simulink model "Mission_Server_QDrone_Manual_Flight_FrSky_FA"  (Simulink 9.3)
settings: Solver=ode2  StartTime=0.0  StopTime=inf  FixedStep=0.001  RelTol=1e-3  EnableMultiTasking=on
InitFcn:
  | addpath(fileparts(get_param(bdroot,'FileName')));setup_project;
undefined symbols (not defined in the file or in its folder): datetime, Host, m, Mission_Server_, saved_data
libraries: quarc_library x16, simulink x5
settings Model: Creator=Admin  LastModifiedBy=user  SimulationMode=external  ExtModeTrigDuration=10000
settings SolverCC: PositivePriorityOrder=on
settings DataIOCC: SaveFormat=Dataset  SignalLoggingSaveFormat=Dataset
settings OptimizationCC: LifeSpan=auto
settings DebuggingCC: UnderspecifiedInitializationDetection=Simplified  MergeDetectMultiDrivingBlocksExec=error  FcnCallInpInsideContextMsg=error
settings HardwareCC: ProdBitPerPointer=64  ProdBitPerSizeT=64  ProdBitPerPtrDiffT=64  ProdLargestAtomicFloat=Float  ProdIntDivRoundTo=Zero  ProdEndianess=LittleEndian  ProdWordSize=64  ProdHWDeviceType=Intel->x86-64 (Windows64)
settings ModelReferenceCC: PropagateSignalLabelsOutOfModel=on
settings RTWCC: SystemTargetFile=quarc_win64.tlc  TemplateMakefile=quarc_default_tmf  Description=QUARC Win64 Target Using Toolchain  Toolchain=QUARC win64 | nmake (64-bit Windows)  BuildConfiguration=Faster Runs
settings STFCustomTargetCC: TargetPreCompLibLocation=C:\PROGRA~3\QUARC\lib\2019a\win64\release  ConcurrentExecutionCompliant=on  SystemTargetFile=quarc_win64.tlc
settings GRTTargetCC: TargetPreCompLibLocation=C:\PROGRA~3\QUARC\lib\2019a\win64\release  ParMdlRefBuildCompliant=off  CompOptLevelCompliant=off  MatFileLogging=off  CPPClassGenCompliant=off  UseToolchainInfoCompliant=off  ExtMode=on  ExtModeMexFile=quarc_comm  ExtModeMexArgs='-w -d %d -uri %u -URI_Host tcpip://192.168.2.5:18001'
settings ConfigComp: CovHtmlReporting=off

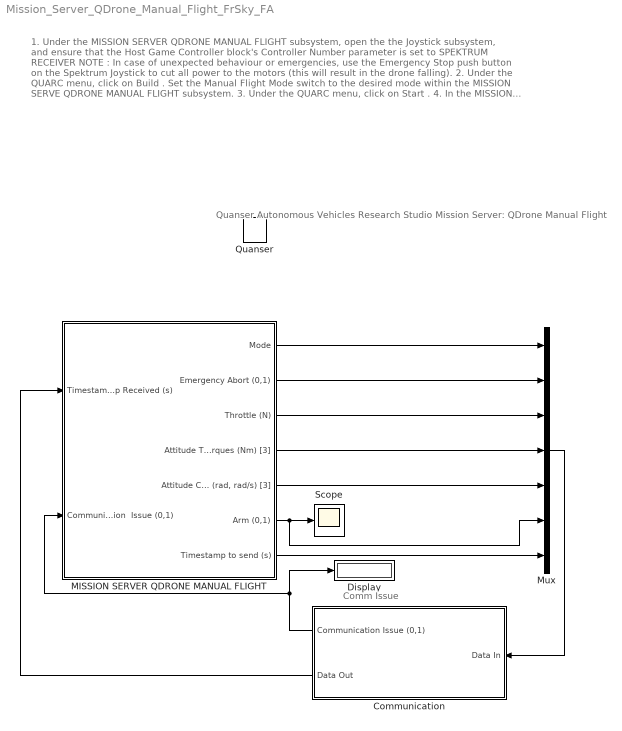
== system Mission_Server_QDrone_Manual_Flight_FrSky_FA ==
  note: Quanser Autonomous Vehicles Research Studio
      | Mission Server: QDrone Manual Flight
  note: 1. Under the MISSION SERVER QDRONE MANUAL FLIGHT subsystem, open the the Joystick subsystem, and ensure that the Host Game Controller block's Controller Number parameter is set to SPEKTRUM RECEIVER
      | NOTE : In case of unexpected behaviour or emergencies, use the Emergency Stop push button on the Spektrum Joystick to cut all power to the motors (this will result in the drone falling).
      | 2. Under the QUARC menu, click on Build . Set the Manual Flight Mode switch to the desired mode within the MISSION SERVE QDRONE MANUAL FLIGHT subsystem.
      | 3. Under the QUARC menu, click on Start .
      | 4. In the MISSION SERVER QDRONE MANUAL FLIGHT subsystem, ensure that the Joystick Issue display shows 0 (joystick must be powered ON with USB dongle attached to the PC).
      | 5. Ensure that the Stabilizer_QDrone.mdl model is running and that the Comm Issue display shows 0.
      | 6. Arm the drone by moving the Arm/Disarm toggle to the 2 position.
      | 7. Fly the drone manually. After landing, move the Arm/Disarm toggle to the 0 position to disarm the QDrone.
      | 8. Stop the Stabilizer_QDrone.mdl model first.
      | 9. Stop this model.
  note: Comm Issue
  Communication : Subsystem
  Display : Display
  MISSION SERVER QDRONE MANUAL FLIGHT : Subsystem
  Mux : Mux  Inputs=7
  Quanser : quarc_library/Logos/Quanser
  Scope : Scope
  wires:
  MISSION SERVER QDRONE MANUAL FLIGHT/7(Timestamp to send (s)) -> Mux/7
  MISSION SERVER QDRONE MANUAL FLIGHT/6(Arm (0,1)) -> Scope/1, Mux/6
  MISSION SERVER QDRONE MANUAL FLIGHT/5("Attitude Commands (rad, rad/s) [3]") -> Mux/5
  Communication/2(Data Out) -> MISSION SERVER QDRONE MANUAL FLIGHT/1(Timestamp Received (s))
  MISSION SERVER QDRONE MANUAL FLIGHT/4(Attitude Torques (Nm) [3]) -> Mux/4
  MISSION SERVER QDRONE MANUAL FLIGHT/3(Throttle (N)) -> Mux/3
  MISSION SERVER QDRONE MANUAL FLIGHT/2(Emergency Abort (0,1)) -> Mux/2
  Mux/1 -> Communication/1(Data In)
  MISSION SERVER QDRONE MANUAL FLIGHT/1(Mode) -> Mux/1
  Communication/1(Communication Issue (0,1)) -> MISSION SERVER QDRONE MANUAL FLIGHT/2(Communication  Issue (0,1)), Display/1

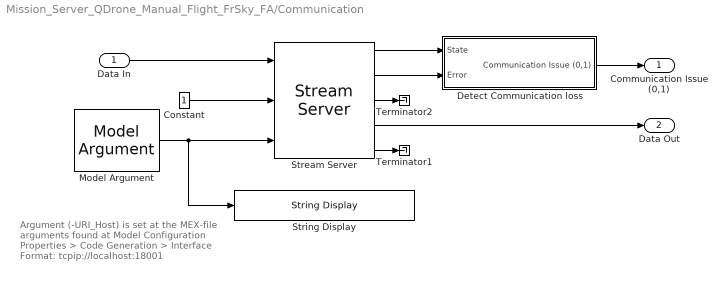
== system Mission_Server_QDrone_Manual_Flight_FrSky_FA/Communication ==
  note: Argument (-URI_Host) is set at the MEX-file arguments found at Model Configuration Properties > Code Generation > Interface
      |
      | Format:
      | tcpip://localhost:18001
  Data In : Inport
  Constant : Constant
  Detect Communication loss : Subsystem
  Model Argument : quarc_library/Sources/Signals/Model Argument  argument_name=URI_Host  has_value=on  data_type_mode=Specify via dialog  data_type=char  max_length=80  variable_size=off
      settings: AttributesFormatString=(-%<argument_name>)  SourceProductName=QUARC Targets
  Stream Server : quarc_library/Communications/Basic/Stream Server  uri_source=External input port  uri=tcpip://localhost:18877  apply_uri_to_all_configs=off  send_buffer_size=1460  receive_buffer_size=1460  byte_order=little endian (Intel - LSB first)  optimization=Minimum latency  send_options=Send most recent data  receive_options=Receive most recent data  default_value=zeros(1,2)  sample_time=qc_get_step_size  active=off  implementation=Use blocking I/O in a separate thread  send_fifo_size=1000  receive_fifo_size=1000  send_priority=0  receive_priority=0  send_dimensions=off  receive_dimensions=off  max_dimensions=-1  data_type=Inherited via back propagation  type_expr=BusObject
  "String Display " : quarc_library/Strings/String Display  alignment=center  display_mode=Single line  sample_time=-1  use_new=off
      settings: SourceProductName=QUARC Targets
  Terminator1 : Terminator
  Terminator2 : Terminator
  Communication Issue (0,1) : Outport
  Data Out : Outport  Port=2
  wires:
  Constant/1 -> Stream Server/2
  Data In/1 -> Stream Server/1
  Stream Server/3 -> Terminator2/1
  Stream Server/5 -> Terminator1/1
  Model Argument/1 -> "String Display "/1, Stream Server/3
  Stream Server/4 -> Data Out/1
  Stream Server/1 -> Detect Communication loss/1(State)
  Stream Server/2 -> Detect Communication loss/2(Error)
  Detect Communication loss/1(Communication Issue (0,1)) -> Communication Issue (0,1)/1

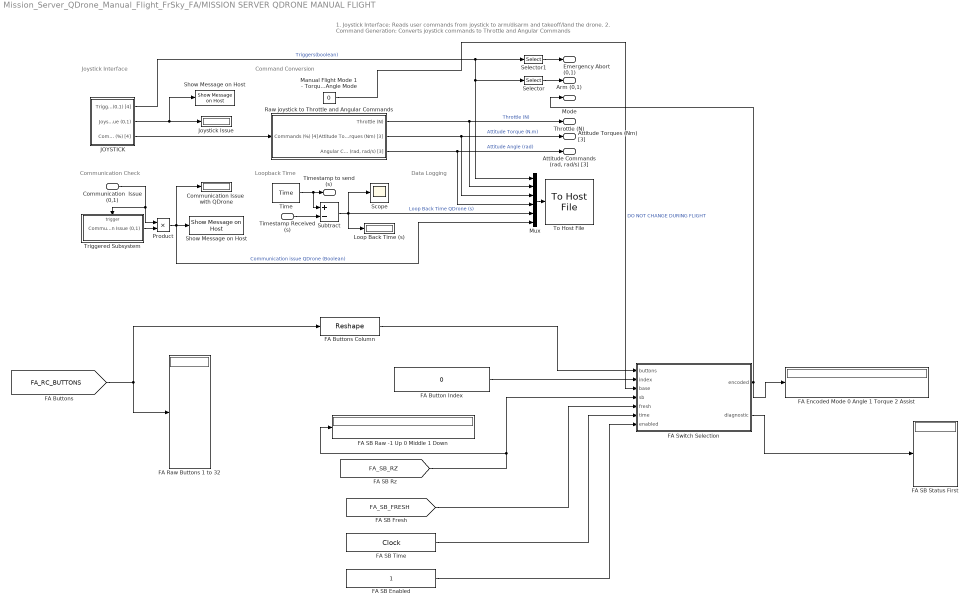
== system Mission_Server_QDrone_Manual_Flight_FrSky_FA/MISSION SERVER QDRONE MANUAL FLIGHT ==
  note: Loopback Time
  note: Command Conversion
  note: Data Logging
  note: Communication Check
  note: Joystick
      | Interface
  note: 1. Joystick Interface: Reads user commands from joystick to arm/disarm and takeoff/land the drone.
      | 2. Command Generation: Converts joystick commands to Throttle and Angular Commands
  Timestamp Received (s) : Inport
  Communication  Issue (0,1) : Inport  Port=2
  Communication Issue  with QDrone : Display
  FA Button Index : Constant  Value=0
  FA Buttons Column : Reshape  OutputDimensionality=Customize  OutputDimensions=[32 1]
  FA Encoded Mode 0 Angle 1 Torque 2 Assist : Display
  FA Raw Buttons 1 to 32 : Display
  FA SB Enabled : Constant
  FA SB Raw -1 Up 0 Middle 1 Down : Display
  FA SB Status First : Display
  FA SB Time : DigitalClock  SampleTime=0.001
  FA Switch Selection : MATLAB Function  TreatAsAtomicUnit=on
  JOYSTICK : Subsystem
  Joystick Issue : Display
  Loop Back Time (s) : Display
  "Manual Flight Mode 1 - Torque Mode,   0 - Angle Mode" : Constant  Value=0
  Mux : Mux  Inputs=6
  Product : Product
  Raw joystick to Throttle and Angular Commands : Subsystem
  Scope : Scope
  Selector : Selector  InputPortWidth=4  IndexOptions=Index vector (dialog)  Indices=[1]  OutputSizes=1
  Selector1 : Selector  InputPortWidth=4  IndexOptions=Index vector (dialog)  Indices=[3]  OutputSizes=1
  Show Message on Host : quarc_library/Sinks/Error Handling/Show Message on Host  message_type=Fixed error message  message_icon=Warning  message=Mission Server: Communication Issue with QDrone
      settings: AttributesFormatString="\"%<message>\""  SourceProductName=QUARC Targets
  "Show Message on Host " : quarc_library/Sinks/Error Handling/Show Message on Host  message_type=Fixed error message  message_icon=Warning  message=Mission Server: Joystick Disconnected
      settings: AttributesFormatString="\"%<message>\""  SourceProductName=QUARC Targets
  Subtract : Sum  Inputs=+-
  Time : quarc_library/Sources/Time/Time  time_source=Wall clock  sample_time=qc_get_step_size
  To Host File : quarc_library/Sinks/To Host/To Host File  file_name=saved_data/%m/Mission_Server_%{char(datetime)}.mat  variable_name=mission_server_data  decimation=1  sample_time=-1  file_format=MAT-file v.5  options=No header or footer  append=off  final_file_name=saved_data/Mission_Server_QDrone_Manual_Flight_FrSky_FA/Mission_Server_10-Nov-2026 20-24-39.mat  bitrate=2000000
  Triggered Subsystem : Subsystem  TreatAsAtomicUnit=on
  Mode : Outport
  Emergency Abort (0,1) : Outport  Port=2
  Throttle (N) : Outport  Port=3
  Attitude Torques (Nm) [3] : Outport  Port=4
  "Attitude Commands (rad, rad/s) [3]" : Outport  Port=5
  Arm (0,1) : Outport  Port=6
  Timestamp to send (s) : Outport  Port=7
  wires:
  Communication  Issue (0,1)/1 -> Product/1, Triggered Subsystem/Trigger
  JOYSTICK/2(Joystick Issue (0,1)) -> "Show Message on Host "/1, Joystick Issue/1
  JOYSTICK/3(Commands (%) [4]) -> Raw joystick to Throttle and Angular Commands/1(Commands (%) [4])
  JOYSTICK/1(Triggers (0,1) [4]) -> Selector1/1, Selector/1, Mux/1  "Triggers(boolean)"
  Time/1 -> Subtract/1, Timestamp to send (s)/1
  Timestamp Received (s)/1 -> Subtract/2
  Subtract/1 -> Loop Back Time (s)/1, Scope/1, Mux/5  "Loop Back Time QDrone (s)"
  Triggered Subsystem/1(Communication Issue (0,1)) -> Product/2
  Product/1 -> Communication Issue  with QDrone/1, Show Message on Host/1, Mux/6  "Communication issue QDrone (Boolean)"
  Mux/1 -> To Host File/1
  Selector/1 -> Arm (0,1)/1
  Selector1/1 -> Emergency Abort (0,1)/1
  Raw joystick to Throttle and Angular Commands/3("Angular Commands (rad, rad/s) [3]") -> "Attitude Commands (rad, rad/s) [3]"/1, Mux/4  "Attitude Angle (rad)"
  Raw joystick to Throttle and Angular Commands/1(Throttle (N)) -> Throttle (N)/1, Mux/2  "Throttle (N)"
  Raw joystick to Throttle and Angular Commands/2(Attitude Torques (Nm) [3]) -> Attitude Torques (Nm) [3]/1, Mux/3  "Attitude Torque (N.m)"
  "Manual Flight Mode 1 - Torque Mode,   0 - Angle Mode"/1 -> FA Switch Selection/3(base)  "DO NOT CHANGE DURING FLIGHT"
  [FA_RC_BUTTONS] -> FA Raw Buttons 1 to 32/1, FA Buttons Column/1
  FA Buttons Column/1 -> FA Switch Selection/1(buttons)
  FA Button Index/1 -> FA Switch Selection/2(index)
  FA Switch Selection/1(encoded) -> FA Encoded Mode 0 Angle 1 Torque 2 Assist/1, Mode/1
  [FA_SB_RZ] -> FA SB Raw -1 Up 0 Middle 1 Down/1, FA Switch Selection/4(sb)
  [FA_SB_FRESH] -> FA Switch Selection/5(fresh)
  FA SB Time/1 -> FA Switch Selection/6(time)
  FA SB Enabled/1 -> FA Switch Selection/7(enabled)
  FA Switch Selection/2(diagnostic) -> FA SB Status First/1

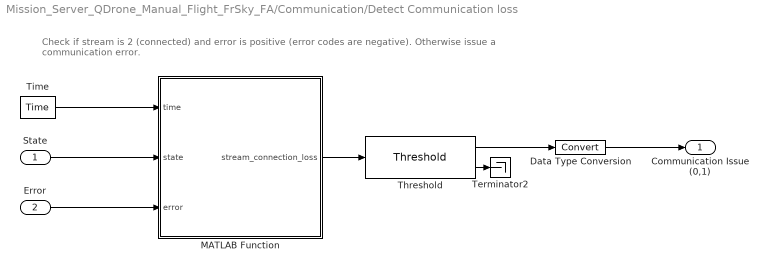
== system Mission_Server_QDrone_Manual_Flight_FrSky_FA/Communication/Detect Communication loss ==
  note: Check if stream is 2 (connected) and error is positive (error codes are negative). Otherwise issue a communication error.
  State : Inport
  Error : Inport  Port=2
  Data Type Conversion : DataTypeConversion
  MATLAB Function : MATLAB Function  TreatAsAtomicUnit=on
  Terminator2 : Terminator
  Threshold : quarc_library/Discontinuities/Threshold  operator=>=  param_src=Specify via dialog  threshold=0.5  duration=0.1
      settings: SourceProductName=QUARC Targets
  Time : quarc_library/Sources/Time/Time  time_source=Wall clock  sample_time=qc_get_step_size
  Communication Issue (0,1) : Outport
  wires:
  Error/1 -> MATLAB Function/3(error)
  MATLAB Function/1(stream_connection_loss) -> Threshold/1
  State/1 -> MATLAB Function/2(state)
  Time/1 -> MATLAB Function/1(time)
  Threshold/2 -> Terminator2/1
  Data Type Conversion/1 -> Communication Issue (0,1)/1
  Threshold/1 -> Data Type Conversion/1

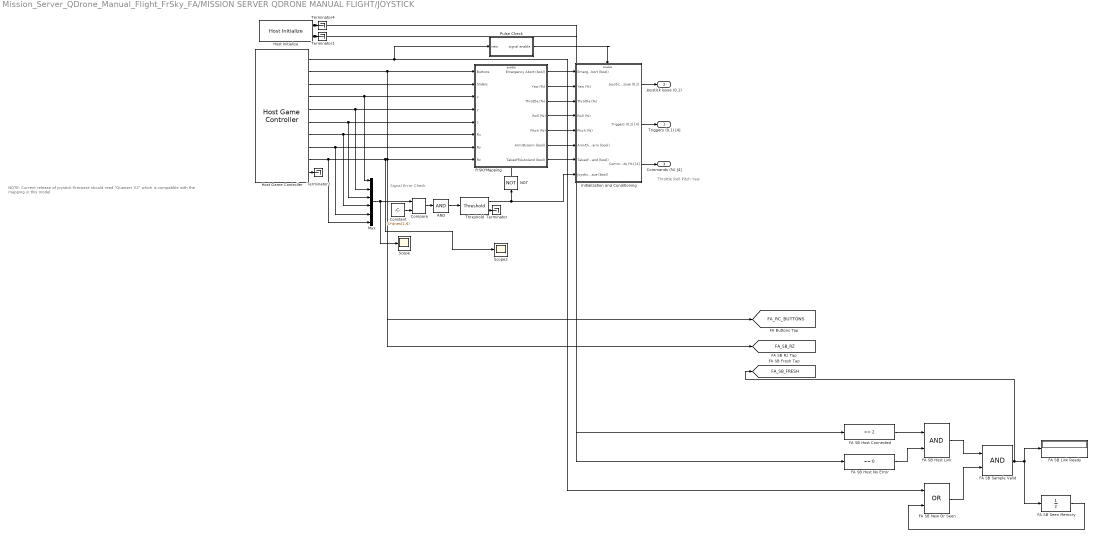
== system Mission_Server_QDrone_Manual_Flight_FrSky_FA/MISSION SERVER QDRONE MANUAL FLIGHT/JOYSTICK ==
  note: Throttle
      | Roll
      | Pitch
      | Yaw
  note: Signal Error Check
  note: NOTE: Current release of joystick firmware should read "Quanser V2" which is compatible with the mapping in this model
  AND : Logic  Inputs=1  AllPortsSameDT=off  OutDataTypeStr=boolean
  Compare : quarc_library/Logic Operations/Compare  operator===  output_data_type=boolean
      settings: SourceProductName=QUARC Targets
  Constant : Constant  Value=-1*ones(1,6)
  FA SB Host Connected : simulink/Logic and Bit Operations/Compare To Constant  relop===  const=2  OutDataTypeStr=boolean
  FA SB Host Link : Logic  AllPortsSameDT=off  OutDataTypeStr=boolean
  FA SB Host No Error : simulink/Logic and Bit Operations/Compare To Constant  relop===  const=0  OutDataTypeStr=boolean
  FA SB Link Ready : Display
  FA SB New Or Seen : Logic  Operator=OR  AllPortsSameDT=off  OutDataTypeStr=boolean
  FA SB Sample Valid : Logic  AllPortsSameDT=off  OutDataTypeStr=boolean
  FA SB Seen Memory : UnitDelay  SampleTime=0.001  HasFrameUpgradeWarning=on
  FrSKYMapping : Subsystem
  Host Game Controller : quarc_library/Devices/Peripherals/Host/Host Game Controller  object_name=Host-1  controller=1  buffer_size=20  deadzone=[]  saturation=[]  sample_time=qc_get_step_size  auto_center=off  enabled=on  debug_mode=off
      settings: SourceProductName=QUARC Targets
  Host Initialize : quarc_library/Devices/Peripherals/Host/Host Initialize  object_name=Host-1  uri_source=Use external mode communications  uri=tcpip://localhost:18001  apply_uri_to_all_configs=on  send_buffer_size=1000  receive_buffer_size=1000  thread_priority=0  run_client=on  use_window=off  window_position=[]  sample_time=qc_get_step_size  active=on
      settings: SourceProductName=QUARC Targets
  Initialization and Conditioning : Subsystem  TreatAsAtomicUnit=on
  Mux : Mux  Inputs=6
  NOT : Logic  Operator=NOT  IconShape=distinctive  AllPortsSameDT=off  OutDataTypeStr=boolean
  Pulse Check : Subsystem  TreatAsAtomicUnit=on
  Scope : Scope
  Scope2 : Scope
  Terminator{,1..2,4} (4 alike) : Terminator
  Threshold : quarc_library/Discontinuities/Threshold  operator=>=  param_src=Specify via dialog  threshold=0.5  duration=0.2
      settings: SourceProductName=QUARC Targets
  Triggers (0,1) [4] : Outport
  Joystick Issue (0,1) : Outport  Port=2
  Commands (%) [4] : Outport  Port=3
  tag scope: FA_RC_BUTTONS=global, FA_SB_FRESH=global, FA_SB_RZ=global
  wires:
  Host Initialize/1 -> Terminator4/1, FA SB Host Connected/1
  Host Initialize/2 -> Terminator1/1, FA SB Host No Error/1
  FrSKYMapping/2(Yaw (%)) -> Initialization and Conditioning/2(Yaw (%))
  FrSKYMapping/3(Throttle (%)) -> Initialization and Conditioning/3(Throttle (%))
  FrSKYMapping/1(Emergency Abort (bool)) -> Initialization and Conditioning/1(Emergency Abort (bool))
  FrSKYMapping/5(Pitch (%)) -> Initialization and Conditioning/5(Pitch (%))
  FrSKYMapping/6("Arm/Disarm (bool) ") -> Initialization and Conditioning/6(Arm/Disarm (bool))
  FrSKYMapping/4(Roll (%)) -> Initialization and Conditioning/4(Roll (%))
  Host Game Controller/1 -> FA SB New Or Seen/1, Pulse Check/1(new)
  Pulse Check/1(signal enable) -> Initialization and Conditioning/Enable
  FrSKYMapping/7(Takeoff/Autoland (bool)) -> Initialization and Conditioning/7(Takeoff/AutoLand (bool))
  Host Game Controller/4 -> Mux/1, FrSKYMapping/3(x)
  Host Game Controller/5 -> Mux/2, FrSKYMapping/4(y)
  Host Game Controller/6 -> Mux/3, FrSKYMapping/5(z)
  Host Game Controller/7 -> Mux/4, FrSKYMapping/6(Rx)
  Host Game Controller/8 -> Mux/5, FrSKYMapping/7(Ry)
  Host Game Controller/9 -> [FA_SB_RZ], FrSKYMapping/8(Rz), Scope2/1, Mux/6
  Mux/1 -> Scope/1, Compare/1
  Constant/1 -> Compare/2
  Compare/1 -> AND/1
  Threshold/2 -> Terminator/1
  Host Game Controller/2 -> FrSKYMapping/1(Buttons), [FA_RC_BUTTONS]
  Host Game Controller/3 -> FrSKYMapping/2(Sliders)
  Threshold/1 -> NOT/1, Initialization and Conditioning/8(Joystick Issue (bool))
  NOT/1 -> FrSKYMapping/Enable
  AND/1 -> Threshold/1
  Initialization and Conditioning/3(Commands (%) [4]) -> Commands (%) [4]/1
  Initialization and Conditioning/2(Triggers (0,1) [4]) -> Triggers (0,1) [4]/1
  Initialization and Conditioning/1(Joystick Issue (0,1)) -> Joystick Issue (0,1)/1
  Host Game Controller/10 -> Terminator2/1
  FA SB Host Connected/1 -> FA SB Host Link/1
  FA SB Host No Error/1 -> FA SB Host Link/2
  FA SB Seen Memory/1 -> FA SB New Or Seen/2
  FA SB Host Link/1 -> FA SB Sample Valid/1
  FA SB New Or Seen/1 -> FA SB Sample Valid/2
  FA SB Sample Valid/1 -> FA SB Seen Memory/1, FA SB Link Ready/1, [FA_SB_FRESH]

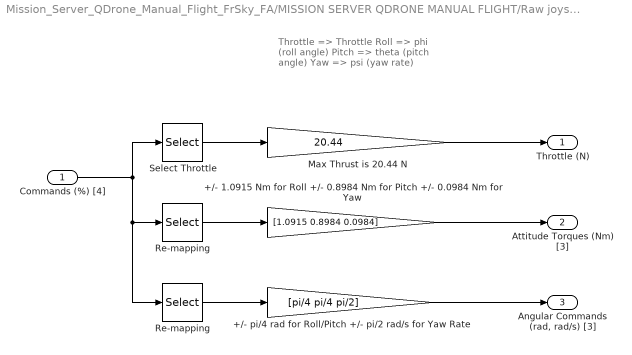
== system Mission_Server_QDrone_Manual_Flight_FrSky_FA/MISSION SERVER QDRONE MANUAL FLIGHT/Raw joystick to Throttle and Angular Commands ==
  note: Throttle 	=> 	 Throttle
      | Roll 	=>	 phi (roll angle)
      | Pitch	=> 	 theta (pitch angle)
      | Yaw		=> 	 psi (yaw rate)
  Commands (%) [4] : Inport
  " Re-mapping " : Selector  InputPortWidth=4  IndexOptions=Index vector (dialog)  Indices=[2 3 4]  OutputSizes=1
  +/- 1.0915 Nm for Roll +/- 0.8984 Nm for Pitch +/- 0.0984 Nm for Yaw : Gain  Gain=[1.0915 0.8984 0.0984]
  +/- pi/4 rad for Roll/Pitch +/- pi/2 rad/s for Yaw Rate : Gain  Gain=[pi/4 pi/4 pi/2]
  Max Thrust is 20.44 N : Gain  Gain=20.44
  Re-mapping : Selector  InputPortWidth=4  IndexOptions=Index vector (dialog)  Indices=[2 3 4]  OutputSizes=1
  Select Throttle : Selector  InputPortWidth=4  IndexOptions=Index vector (dialog)  Indices=[1]  OutputSizes=1
  Throttle (N) : Outport
  Attitude Torques (Nm) [3] : Outport  Port=2
  "Angular Commands (rad, rad/s) [3]" : Outport  Port=3
  wires:
  +/- pi/4 rad for Roll/Pitch +/- pi/2 rad/s for Yaw Rate/1 -> "Angular Commands (rad, rad/s) [3]"/1
  Commands (%) [4]/1 -> Re-mapping/1, " Re-mapping "/1, Select Throttle/1
  Re-mapping/1 -> +/- pi/4 rad for Roll/Pitch +/- pi/2 rad/s for Yaw Rate/1
  Select Throttle/1 -> Max Thrust is 20.44 N/1
  Max Thrust is 20.44 N/1 -> Throttle (N)/1
  " Re-mapping "/1 -> +/- 1.0915 Nm for Roll +/- 0.8984 Nm for Pitch +/- 0.0984 Nm for Yaw/1
  +/- 1.0915 Nm for Roll +/- 0.8984 Nm for Pitch +/- 0.0984 Nm for Yaw/1 -> Attitude Torques (Nm) [3]/1

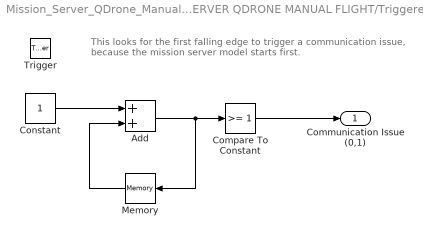
== system Mission_Server_QDrone_Manual_Flight_FrSky_FA/MISSION SERVER QDRONE MANUAL FLIGHT/Triggered Subsystem ==
  note: This looks for the first falling edge to trigger a communication issue,
      | because the mission server model starts first.
  Trigger : TriggerPort  TriggerType=falling  VariantControl=Variant
  Add : Sum
  Compare To Constant : simulink/Logic and Bit Operations/Compare To Constant  relop=>=  const=1  OutDataTypeStr=boolean
  Constant : Constant
  Memory : Memory  InheritSampleTime=on
  Communication Issue (0,1) : Outport  InitialOutput=0
  wires:
  Constant/1 -> Add/1
  Memory/1 -> Add/2
  Add/1 -> Compare To Constant/1, Memory/1
  Compare To Constant/1 -> Communication Issue (0,1)/1

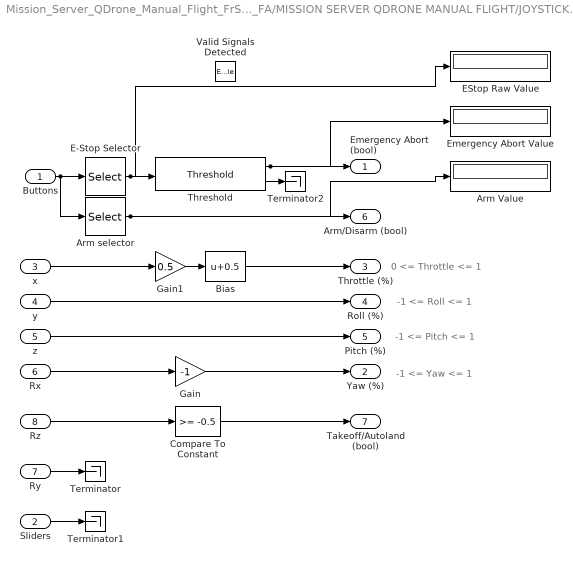
== system Mission_Server_QDrone_Manual_Flight_FrSky_FA/MISSION SERVER QDRONE MANUAL FLIGHT/JOYSTICK/FrSKYMapping ==
  note: -1 <= Yaw <= 1
  note: 0 <= Throttle <= 1
  note: -1 <= Roll <= 1
  note: -1 <= Pitch <= 1
  Buttons : Inport
  Sliders : Inport  Port=2
  x : Inport  Port=3
  y : Inport  Port=4
  z : Inport  Port=5
  Rx : Inport  Port=6
  Ry : Inport  Port=7
  Rz : Inport  Port=8
  Valid Signals Detected : EnablePort
  Arm Value : Display
  Arm selector : Selector  InputPortWidth=32  IndexOptions=Index vector (dialog)  Indices=[2]  OutputSizes=1
  Bias : Bias  Bias=0.5
  Compare To Constant : simulink/Logic and Bit Operations/Compare To Constant  relop=>=  const=-0.5  OutDataTypeStr=boolean
  E-Stop Selector : Selector  InputPortWidth=32  IndexOptions=Index vector (dialog)  Indices=[1]  OutputSizes=1
  EStop Raw Value : Display
  Emergency Abort Value : Display
  Gain : Gain  Gain=-1
  Gain1 : Gain  Gain=0.5
  Terminator : Terminator
  Terminator1 : Terminator
  Terminator2 : Terminator
  Threshold : quarc_library/Discontinuities/Threshold  operator=>=  param_src=Specify via dialog  threshold=0.5  duration=0.2
      settings: SourceProductName=QUARC Targets
  Emergency Abort (bool) : Outport
  Yaw (%) : Outport  Port=2
  Throttle (%) : Outport  Port=3
  Roll (%) : Outport  Port=4
  Pitch (%) : Outport  Port=5
  "Arm/Disarm (bool) " : Outport  Port=6
  Takeoff/Autoland (bool) : Outport  Port=7
  wires:
  Buttons/1 -> Arm selector/1, E-Stop Selector/1
  Arm selector/1 -> "Arm/Disarm (bool) "/1, Arm Value/1
  x/1 -> Gain1/1
  y/1 -> Roll (%)/1
  z/1 -> Pitch (%)/1
  Rx/1 -> Gain/1
  Ry/1 -> Terminator/1
  Sliders/1 -> Terminator1/1
  E-Stop Selector/1 -> Threshold/1, EStop Raw Value/1
  Rz/1 -> Compare To Constant/1
  Compare To Constant/1 -> Takeoff/Autoland (bool)/1
  Threshold/1 -> Emergency Abort (bool)/1, Emergency Abort Value/1
  Threshold/2 -> Terminator2/1
  Gain/1 -> Yaw (%)/1
  Gain1/1 -> Bias/1
  Bias/1 -> Throttle (%)/1

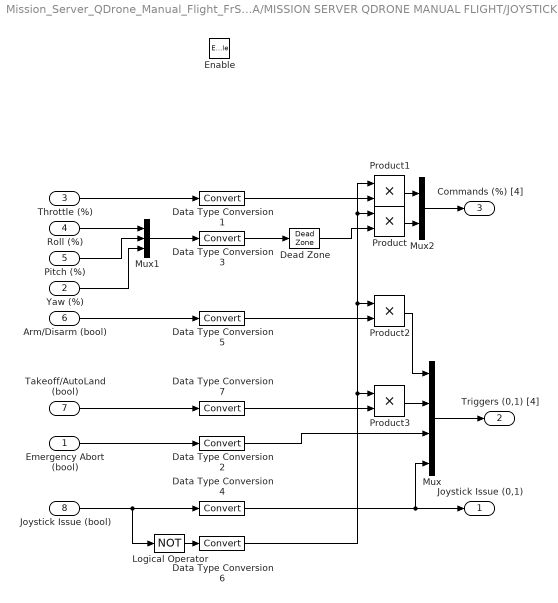
== system Mission_Server_QDrone_Manual_Flight_FrSky_FA/MISSION SERVER QDRONE MANUAL FLIGHT/JOYSTICK/Initialization and Conditioning ==
  Emergency Abort (bool) : Inport
  Yaw (%) : Inport  Port=2
  Throttle (%) : Inport  Port=3
  Roll (%) : Inport  Port=4
  Pitch (%) : Inport  Port=5
  Arm/Disarm (bool) : Inport  Port=6
  Takeoff/AutoLand (bool) : Inport  Port=7
  Joystick Issue (bool) : Inport  Port=8
  Enable : EnablePort  StatesWhenEnabling=reset
  Data Type Conversion{1..7} (7 alike) : DataTypeConversion
  Dead Zone : DeadZone  LowerValue=[-0.01 -0.02 -0.01]  UpperValue=[0.01 0.02 0.01]  SaturateOnIntegerOverflow=on
  Logical Operator : Logic  Operator=NOT  AllPortsSameDT=off  OutDataTypeStr=boolean
  Mux : Mux
  Mux1 : Mux  Inputs=3
  Mux2 : Mux  Inputs=2
  Product{,1..3} (4 alike) : Product
  Joystick Issue (0,1) : Outport  InitialOutput=0
  Triggers (0,1) [4] : Outport  Port=2  InitialOutput=0
  Commands (%) [4] : Outport  Port=3  InitialOutput=0
  wires:
  Joystick Issue (bool)/1 -> Data Type Conversion4/1, Logical Operator/1
  Mux1/1 -> Data Type Conversion3/1
  Throttle (%)/1 -> Data Type Conversion1/1
  Roll (%)/1 -> Mux1/1
  Pitch (%)/1 -> Mux1/2
  Yaw (%)/1 -> Mux1/3
  Data Type Conversion4/1 -> Mux/4, Joystick Issue (0,1)/1
  Emergency Abort (bool)/1 -> Data Type Conversion2/1
  Data Type Conversion3/1 -> Dead Zone/1
  Arm/Disarm (bool)/1 -> Data Type Conversion5/1
  Mux/1 -> Triggers (0,1) [4]/1
  Data Type Conversion2/1 -> Mux/3
  Logical Operator/1 -> Data Type Conversion6/1
  Product/1 -> Mux2/2
  Product1/1 -> Mux2/1
  Data Type Conversion1/1 -> Product1/2
  Dead Zone/1 -> Product/2
  Data Type Conversion6/1 -> Product1/1, Product/1, Product2/1, Product3/1
  Product2/1 -> Mux/1
  Data Type Conversion5/1 -> Product2/2
  Takeoff/AutoLand (bool)/1 -> Data Type Conversion7/1
  Product3/1 -> Mux/2
  Data Type Conversion7/1 -> Product3/2
  Mux2/1 -> Commands (%) [4]/1

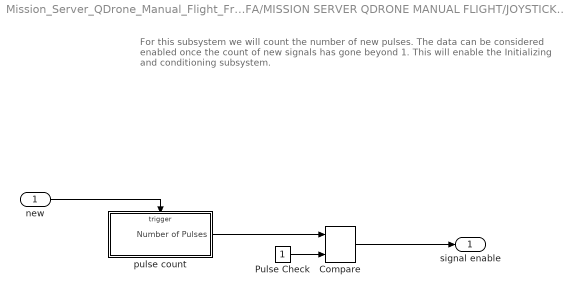
== system Mission_Server_QDrone_Manual_Flight_FrSky_FA/MISSION SERVER QDRONE MANUAL FLIGHT/JOYSTICK/Pulse Check ==
  note: For this subsystem we will count the number of new pulses. The data can be considered enabled once the count of new signals has gone beyond 1. This will enable the Initializing and conditioning subsystem.
  new : Inport
  Compare : quarc_library/Logic Operations/Compare  operator=>=  output_data_type=boolean
      settings: SourceProductName=QUARC Targets
  Pulse Check : Constant
  "pulse count " : Subsystem  TreatAsAtomicUnit=on
  signal enable : Outport  InitialOutput=0
  wires:
  Compare/1 -> signal enable/1
  Pulse Check/1 -> Compare/2
  new/1 -> "pulse count "/Trigger
  "pulse count "/1(Number of Pulses) -> Compare/1

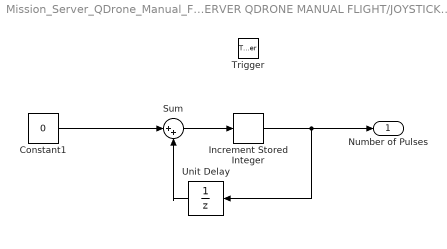
== system Mission_Server_QDrone_Manual_Flight_FrSky_FA/MISSION SERVER QDRONE MANUAL FLIGHT/JOYSTICK/Pulse Check/pulse count  ==
  Trigger : TriggerPort  TriggerType=either  VariantControl=Variant
  Constant1 : Constant  Value=0
  Increment Stored Integer : simulink/Additional Math & Discrete/Additional Math: Increment - Decrement/Increment Stored Integer
  Sum : Sum  Inputs=|++
  Unit Delay : UnitDelay  SampleTime=-1  HasFrameUpgradeWarning=on
  Number of Pulses : Outport
  wires:
  Constant1/1 -> Sum/1
  Sum/1 -> Increment Stored Integer/1
  Unit Delay/1 -> Sum/2
  Increment Stored Integer/1 -> Unit Delay/1, Number of Pulses/1

== matlab function MISSION SERVER QDRONE MANUAL FLIGHT/FA Switch Selection ==
  settings: updateMethod=DISCRETE  sampleTime=0.001
  data: buttons input double size=[32 1]; encoded output double size=1; index input double size=1; base input double size=1; sb input double size=1; fresh input double size=1; time input double size=1; enabled input double size=1; diagnostic output double size=[6 1]
function [encoded,diagnostic]=select(buttons,index,base,sb,fresh,time,enabled)
%#codegen
% buttons/index retained only to preserve the original input connections.
[encoded,diagnostic]=qdrone_sb_mode_step(sb,fresh,time,base,enabled);
end

== matlab function Communication/Detect Communication loss/MATLAB Function ==
  data: time input double; stream_connection_loss output double; state input double; error input double
function stream_connection_loss  = fcn(time, state, error)

stream_connection_loss = 0;
if time > 1
    if ~((state == 2)&&(error >= 0))
        % stream connection is not established correctly
        stream_connection_loss = 1;
    end
end
